simulink model "AFC_FFNN_trainbfg_15_15_15_15_Nor_July_15_RepFast"  (R2021a)
settings: Solver=ode15s  StartTime=0.0  StopTime=T  MaxStep=.01  RelTol=1e-3
undefined symbols (not defined in the file): AF_sensor_tol, fault_time, fuel_inj_tol, kappa_tol, MAF_sensor_tol, patch_sig, pump_tol, safe_patch_sig, sw, tau_ww_tol, x_gain, x_offset, y_gain, y_offset
libraries: neural x66, simulink x3
(part 1 of 3)
Description:
  | Modeling Engine Timing Using Triggered Subsystems
  | 
  | This example presents a model of a four-cylinder spark ignition engine
  | and demonstrates Simulink(R) capabilities to model an internal combustion
  | engine from the throttle to the crankshaft output. We used well-defined
  | physical principles supplemented, where appropriate, with empirical
  | relationships that describe the systems dynamic behavior without
  | introducing unnecessary complexity.
settings Model: SimulationMode=accelerator  ExtModeTrigMode=oneshot  ExtModeArmWhenConnect=off  ExtModeAutoUpdateStatusClock=off  Creator=The MathWorks Inc.  LastModifiedBy=deyun
settings SolverCC: ZeroCrossControl=DisableAll  AlgebraicLoopSolver=TrustRegion
settings DataIOCC: ExternalInput=[t__, u__]  LoadExternalInput=on  SaveFormat=StructureWithTime  SignalLogging=off  DSMLogging=off  ReturnWorkspaceOutputs=off
settings OptimizationCC: BlockReduction=off  BooleanDataType=off  LifeSpan=inf
settings DebuggingCC: SaveWithParameterizedLinksMsg=none  UnderspecifiedInitializationDetection=Classic  MergeDetectMultiDrivingBlocksExec=none  SignalResolutionControl=TryResolveAllWithWarning  ParameterPrecisionLossMsg=none  SFUnexpectedBacktrackingDiag=warning  SFNoUnconditionalDefaultTransitionDiag=warning  SFExecutionAtInitializationDiag=none  ArithmeticOperatorsInVariantConditions=warning
settings HardwareCC: ProdBitPerPointer=32  ProdBitPerSizeT=32  ProdBitPerPtrDiffT=32  ProdLargestAtomicFloat=None  ProdIntDivRoundTo=Undefined  ProdEndianess=Unspecified  ProdWordSize=32  ProdHWDeviceType=32-bit Generic  TargetBitPerLong=64  TargetBitPerPointer=64  TargetBitPerSizeT=64  TargetBitPerPtrDiffT=64  TargetLongLongMode=on  TargetIntDivRoundTo=Zero  TargetEndianess=LittleEndian  TargetWordSize=64  TargetHWDeviceType=MATLAB Host  ProdEqTarget=off
settings ModelReferenceCC: PropagateSignalLabelsOutOfModel=off
settings SFSimCC: SimUseLocalCustomCode=off  CustomCodeUndefinedFunction=UseInterfaceOnly
settings RTWCC: RTWUseLocalCustomCode=off
settings CodeAppCC: StateflowObjectComments=on
settings GRTTargetCC: TargetLangStandard=C89/C90 (ANSI)
settings ConfigComp: CovMetricSettings=d  CovSaveCumulativeToWorkspaceVar=on  CovSaveSingleToWorkspaceVar=on  CovExternalEMLEnable=off  CovBoundaryAbsTol=1.0e-5

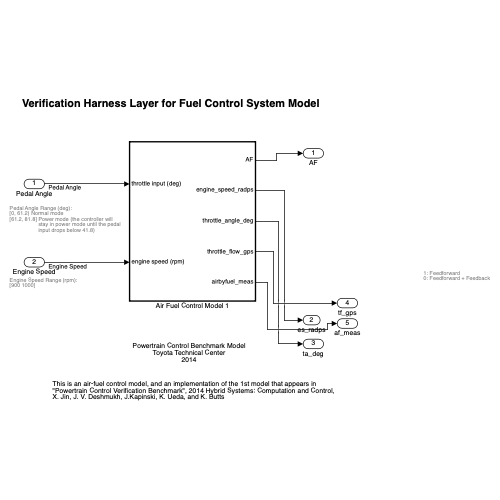
[thumbnail: Simulink's stored preview of the top-level diagram]
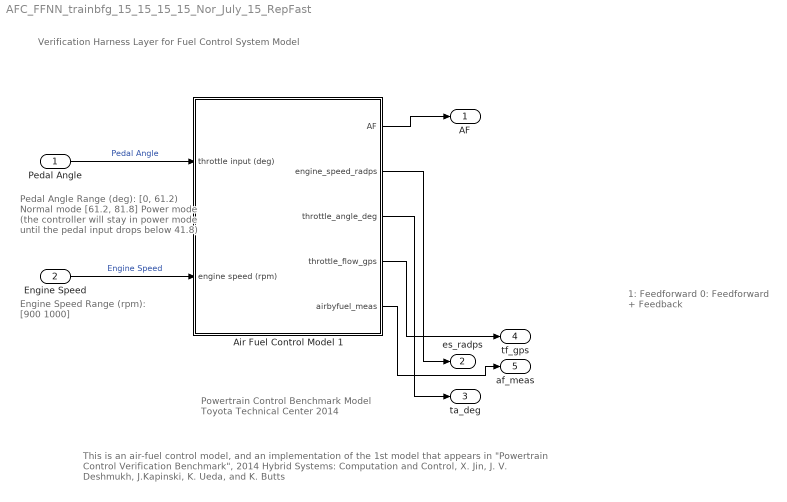
== system AFC_FFNN_trainbfg_15_15_15_15_Nor_July_15_RepFast ==
  note: 1: Feedforward
      | 0: Feedforward + Feedback
  note: Pedal Angle Range (deg):
      | [0, 61.2) Normal mode
      | [61.2, 81.8] Power mode (the controller will
      |                    stay in power mode until the pedal
      |                    input drops below 41.8)
  note: This is an air-fuel control model, and an implementation of the 1st model that appears in
      | "Powertrain Control Verification Benchmark", 2014 Hybrid Systems: Computation and Control,
      | X. Jin, J. V. Deshmukh, J.Kapinski, K. Ueda, and K. Butts
  note: Engine Speed Range (rpm):
      | [900 1000]
  note: Powertrain Control Benchmark Model
      | Toyota Technical Center
      | 2014
  note: Verification Harness Layer for Fuel Control System Model
  Pedal Angle : Inport  Interpolate=off
  Engine Speed : Inport  Port=2  Interpolate=off
  Air Fuel Control Model 1 : Subsystem  Priority=1  TreatAsAtomicUnit=on
  AF : Outport  VectorParamsAs1DForOutWhenUnconnected=off
  es_radps : Outport  Port=2
  ta_deg : Outport  Port=3
  tf_gps : Outport  Port=4
  af_meas : Outport  Port=5
  wires:
  Air Fuel Control Model 1/1(AF) -> AF/1
  Pedal Angle/1 -> Air Fuel Control Model 1/1(throttle input (deg))  "Pedal Angle"
  Engine Speed/1 -> Air Fuel Control Model 1/2(engine speed (rpm))  "Engine Speed"
  Air Fuel Control Model 1/2(engine_speed_radps) -> es_radps/1
  Air Fuel Control Model 1/3(throttle_angle_deg) -> ta_deg/1
  Air Fuel Control Model 1/4(throttle_flow_gps) -> tf_gps/1
  Air Fuel Control Model 1/5(airbyfuel_meas) -> af_meas/1

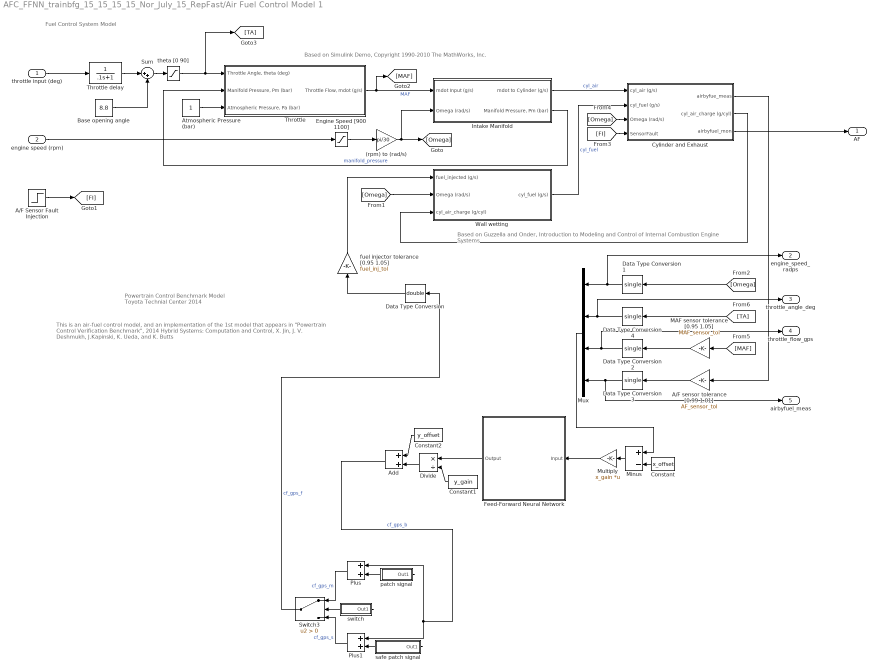
== system AFC_FFNN_trainbfg_15_15_15_15_Nor_July_15_RepFast/Air Fuel Control Model 1 ==
  note: Based on Simulink Demo, Copyright 1990-2010 The MathWorks, Inc.
  note: Based on Guzzella and Onder, Introduction to Modeling and Control of Internal Combustion Engine Systems
  note: Fuel Control System Model
  note: This is an air-fuel control model, and an implementation of the 1st model that appears in
      | "Powertrain Control Verification Benchmark", 2014 Hybrid Systems: Computation and Control,
      | X. Jin, J. V. Deshmukh, J.Kapinski, K. Ueda, and K. Butts
  note: Powertrain Control Benchmark Model
      | Toyota Technial Center
      | 2014
  throttle input (deg) : Inport  Description=[0, 81.2]
      settings: AttributesFormatString=%<Description>
  engine speed (rpm) : Inport  Description=[900,1100]  Port=2
      settings: AttributesFormatString=%<Description>
  (rpm) to (rad/s) : Gain  Gain=pi/30
  A/F Sensor Fault Injection : Step  Time=fault_time  SampleTime=0
      settings: AttributesFormatString=1: Failure\n0: Normal
  A/F sensor tolerance [0.99 1.01] : Gain  Gain=AF_sensor_tol
  Add : Sum
  Atmospheric Pressure (bar) : Constant
  Base opening angle : Constant  Value=8.8
  Constant : Constant  Value=x_offset
  Constant1 : Constant  Value=y_gain
  Constant2 : Constant  Value=y_offset
  Cylinder and Exhaust : Subsystem
  Data Type Conversion : DataTypeConversion  OutDataTypeStr=double
  Data Type Conversion{1..4} (4 alike) : DataTypeConversion  OutDataTypeStr=single
  Divide : Product  Inputs=*/
  Engine Speed [900 1100] : Saturate  UpperLimit=1100  LowerLimit=900
  Feed-Forward Neural Network : Subsystem
      mask help: Feed-Forward Neural Network
      mask Display: e = 0.06;c1 = [120 150 230]/255;c2 = ([120 150 230]+0)/383;c3 = ([120 150 230]+128)/383;patch([0 1 1 0],[0 0 1 1],c1);patch([0 1 1 1-e 1-e 0+e],[0 0 1 1-e 0+e 0+e],c2);patch([0 0 1 1-e 0+e 0+e],[0 1 1 1-e 1-e 0+e],c3);plot([0 1 1 0 0],[0 0 1 1 0]);fprintf('NNET');port_label('input',1,' Input');port_label('output',1,'Output ');
  Intake Manifold : Subsystem
  MAF sensor tolerance [0.95 1.05] : Gain  Gain=MAF_sensor_tol
  Minus : Sum  Inputs=+-
  Multiply : Gain  Gain=x_gain  Multiplication=Matrix(K*u)
  Mux : Mux
  Plus : Sum
  Plus1 : Sum
  Sum : Sum  Inputs=|++
  Switch3 : Switch  Criteria=u2 > Threshold
  Throttle : Subsystem
  Throttle delay : TransferFcn  Denominator=[.1 1]
  Wall wetting : Subsystem
  fuel injector tolerance [0.95 1.05] : Gain  Gain=fuel_inj_tol
  patch signal : Subsystem
  safe patch signal : Subsystem
  switch : Subsystem
  theta [0 90] : Saturate  UpperLimit=90  LowerLimit=0
  AF : Outport  VectorParamsAs1DForOutWhenUnconnected=off
  engine_speed_radps : Outport  Port=2
  throttle_angle_deg : Outport  Port=3
  throttle_flow_gps : Outport  Port=4
  airbyfuel_meas : Outport  Port=5
  wires:
  (rpm) to (rad/s)/1 -> [Omega], Intake Manifold/2(Omega (rad/s))
  Data Type Conversion/1 -> fuel injector tolerance [0.95 1.05]/1
  theta [0 90]/1 -> Throttle/1("Throttle Angle, theta (deg)"), [TA]
  Engine Speed [900 1100]/1 -> (rpm) to (rad/s)/1
  Cylinder and Exhaust/3("airbyfuel_mon ") -> AF/1
  A/F sensor tolerance [0.99 1.01]/1 -> Data Type Conversion3/1
  [MAF] -> MAF sensor tolerance [0.95 1.05]/1
  Cylinder and Exhaust/1(airbyfue_meas) -> A/F sensor tolerance [0.99 1.01]/1
  Throttle/1("Throttle Flow, mdot (g/s)") -> [MAF], Intake Manifold/1(mdot Input (g/s))  "MAF"
  Intake Manifold/2("Manifold Pressure, Pm (bar)") -> Throttle/2("Manifold Pressure, Pm (bar)")  "manifold_pressure"
  Atmospheric Pressure (bar)/1 -> Throttle/3("Atmospheric Pressure, Pa (bar) ")
  Wall wetting/1(cyl_fuel (g/s)) -> Cylinder and Exhaust/2(cyl_fuel (g/s))  "cyl_fuel"
  Intake Manifold/1(mdot to Cylinder (g/s)) -> Cylinder and Exhaust/1(cyl_air (g/s))  "cyl_air"
  [Omega] -> Cylinder and Exhaust/3(Omega (rad/s))
  [Omega] -> Wall wetting/2(Omega (rad/s))
  Cylinder and Exhaust/2(cyl_air_charge (g/cyl)) -> Wall wetting/3(cyl_air_charge (g/cyl))
  [Omega] -> Data Type Conversion1/1
  fuel injector tolerance [0.95 1.05]/1 -> Wall wetting/1(fuel_injected (g/s))
  MAF sensor tolerance [0.95 1.05]/1 -> Data Type Conversion2/1
  A/F Sensor Fault Injection/1 -> [FI]
  [FI] -> Cylinder and Exhaust/4(SensorFault)
  [TA] -> Data Type Conversion4/1
  throttle input (deg)/1 -> Throttle delay/1
  engine speed (rpm)/1 -> Engine Speed [900 1100]/1
  Throttle delay/1 -> Sum/1
  Base opening angle/1 -> Sum/2
  Sum/1 -> theta [0 90]/1
  Data Type Conversion3/1 -> airbyfuel_meas/1, Mux/4
  Data Type Conversion4/1 -> Mux/2, throttle_angle_deg/1
  Data Type Conversion2/1 -> Mux/3, throttle_flow_gps/1
  Data Type Conversion1/1 -> Mux/1, engine_speed_radps/1
  Multiply/1 -> Feed-Forward Neural Network/1(Input)
  Constant/1 -> Minus/2
  Mux/1 -> Minus/1
  Minus/1 -> Multiply/1
  Constant2/1 -> Add/1
  Feed-Forward Neural Network/1(Output) -> Divide/1
  Constant1/1 -> Divide/2
  Divide/1 -> Add/2
  Plus1/1 -> Switch3/3  "cf_gps_s"
  Switch3/1 -> Data Type Conversion/1  "cf_gps_f"
  Add/1 -> Plus/1, Plus1/1  "cf_gps_b"
  Plus/1 -> Switch3/1  "cf_gps_m"
  patch signal/1(Out1) -> Plus/2
  safe patch signal/1(Out1) -> Plus1/2
  switch/1(Out1) -> Switch3/2

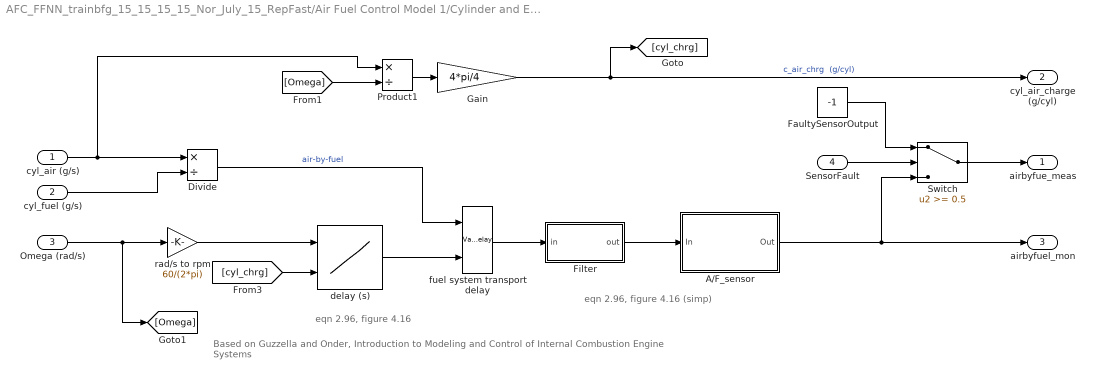
== system AFC_FFNN_trainbfg_15_15_15_15_Nor_July_15_RepFast/Air Fuel Control Model 1/Cylinder and Exhaust ==
  note: Based on Guzzella and Onder, Introduction to Modeling and Control of Internal Combustion Engine Systems
  note: eqn 2.96, figure 4.16
  note: eqn 2.96, figure 4.16 (simp)
  cyl_air (g/s) : Inport
  cyl_fuel (g/s) : Inport  Port=2
  Omega (rad/s) : Inport  Port=3
  SensorFault : Inport  Port=4
  A/F_sensor : Subsystem
  Divide : Product  Inputs=*/
  FaultySensorOutput : Constant  Value=-1
  Filter : Subsystem
  Gain : Gain  Gain=4*pi/4
  Product1 : Product  Inputs=*/  RndMeth=Zero
  Switch : Switch  Threshold=0.5
  delay (s) : Lookup_n-D  BreakpointsForDimension1=[800,1000,1500,2000,3000]  BreakpointsForDimension2=[0.05,0.15,0.2,0.25]  Table=reshape([0.8,0.6,0.4,0.3,0.2,0.4,0.3,0.2,0.2,0.2,0.3,0.25,0.2,0.2,0.2,0.25,0.2,0.2,0.2,0.2],5,4)  UseLastTableValue=on  RndMeth=Simplest  InputSameDT=on
      settings: InputPortMap=u0,u1
  fuel system transport delay : VariableTransportDelay  VariableDelayType=Variable transport delay  MaximumDelay=10  InitialOutput=14.7  MaximumPoints=20480
  rad/s to rpm : Gain  Gain=60/(2*pi)
  airbyfue_meas : Outport  VectorParamsAs1DForOutWhenUnconnected=off
  cyl_air_charge (g/cyl) : Outport  Port=2  VectorParamsAs1DForOutWhenUnconnected=off
  "airbyfuel_mon " : Outport  Port=3  VectorParamsAs1DForOutWhenUnconnected=off
  wires:
  cyl_air (g/s)/1 -> Divide/1, Product1/1
  [Omega] -> Product1/2
  Product1/1 -> Gain/1
  Gain/1 -> [cyl_chrg], cyl_air_charge (g/cyl)/1  "c_air_chrg  (g/cyl)"
  [cyl_chrg] -> delay (s)/2
  cyl_fuel (g/s)/1 -> Divide/2
  Omega (rad/s)/1 -> [Omega], rad/s to rpm/1
  rad/s to rpm/1 -> delay (s)/1
  delay (s)/1 -> fuel system transport delay/2
  fuel system transport delay/1 -> Filter/1(in)
  Switch/1 -> airbyfue_meas/1
  Divide/1 -> fuel system transport delay/1  "air-by-fuel"
  Filter/1(out) -> A/F_sensor/1(In)
  FaultySensorOutput/1 -> Switch/1
  SensorFault/1 -> Switch/2
  A/F_sensor/1(Out) -> Switch/3, "airbyfuel_mon "/1

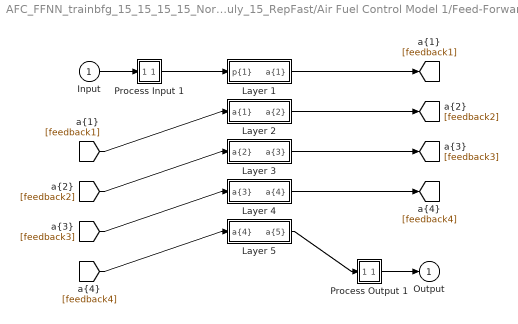
== system AFC_FFNN_trainbfg_15_15_15_15_Nor_July_15_RepFast/Air Fuel Control Model 1/Feed-Forward Neural Network ==
  Input : Inport  PortDimensions=4
      mask Display: e = 0.06;c1 = [120 230 180]/255;c2 = ([120 230 180]+0)/(256+128);c3 = ([120 230 180]+128)/(256+128);patch([0 1 1 0],[0 0 1 1],c1);patch([0 1 1 1-e 1-e 0+e],[0 0 1 1-e 0+e 0+e],c2);patch([0 0 1 1-e 0+e 0+e],[0 1 1 1-e 1-e 0+e],c3);plot([0 1 1 0 0],[0 0 1 1 0]);
  Layer 1 : Subsystem
      mask Display: e = 0.06;c1 = [120 150 230]/255;c2 = ([120 150 230]+0)/383;c3 = ([120 150 230]+128)/383;patch([0 1 1 0],[0 0 1 1],c1);patch([0 1 1 1-e 1-e 0+e],[0 0 1 1-e 0+e 0+e],c2);patch([0 0 1 1-e 0+e 0+e],[0 1 1 1-e 1-e 0+e],c3);plot([0 1 1 0 0],[0 0 1 1 0]);
  Layer 2 : Subsystem
      mask Display: e = 0.06;c1 = [120 150 230]/255;c2 = ([120 150 230]+0)/383;c3 = ([120 150 230]+128)/383;patch([0 1 1 0],[0 0 1 1],c1);patch([0 1 1 1-e 1-e 0+e],[0 0 1 1-e 0+e 0+e],c2);patch([0 0 1 1-e 0+e 0+e],[0 1 1 1-e 1-e 0+e],c3);plot([0 1 1 0 0],[0 0 1 1 0]);
  Layer 3 : Subsystem
      mask Display: e = 0.06;c1 = [120 150 230]/255;c2 = ([120 150 230]+0)/383;c3 = ([120 150 230]+128)/383;patch([0 1 1 0],[0 0 1 1],c1);patch([0 1 1 1-e 1-e 0+e],[0 0 1 1-e 0+e 0+e],c2);patch([0 0 1 1-e 0+e 0+e],[0 1 1 1-e 1-e 0+e],c3);plot([0 1 1 0 0],[0 0 1 1 0]);
  Layer 4 : Subsystem
      mask Display: e = 0.06;c1 = [120 150 230]/255;c2 = ([120 150 230]+0)/383;c3 = ([120 150 230]+128)/383;patch([0 1 1 0],[0 0 1 1],c1);patch([0 1 1 1-e 1-e 0+e],[0 0 1 1-e 0+e 0+e],c2);patch([0 0 1 1-e 0+e 0+e],[0 1 1 1-e 1-e 0+e],c3);plot([0 1 1 0 0],[0 0 1 1 0]);
  Layer 5 : Subsystem
      mask Display: e = 0.06;c1 = [120 150 230]/255;c2 = ([120 150 230]+0)/383;c3 = ([120 150 230]+128)/383;patch([0 1 1 0],[0 0 1 1],c1);patch([0 1 1 1-e 1-e 0+e],[0 0 1 1-e 0+e 0+e],c2);patch([0 0 1 1-e 0+e 0+e],[0 1 1 1-e 1-e 0+e],c3);plot([0 1 1 0 0],[0 0 1 1 0]);
  Process Input 1 : Subsystem
      mask Display: e = 0.06;c1 = [120 150 230]/255;c2 = ([120 150 230]+0)/383;c3 = ([120 150 230]+128)/383;patch([0 1 1 0],[0 0 1 1],c1);patch([0 1 1 1-e 1-e 0+e],[0 0 1 1-e 0+e 0+e],c2);patch([0 0 1 1-e 0+e 0+e],[0 1 1 1-e 1-e 0+e],c3);plot([0 1 1 0 0],[0 0 1 1 0]);
  Process Output 1 : Subsystem
      mask Display: e = 0.06;c1 = [120 150 230]/255;c2 = ([120 150 230]+0)/383;c3 = ([120 150 230]+128)/383;patch([0 1 1 0],[0 0 1 1],c1);patch([0 1 1 1-e 1-e 0+e],[0 0 1 1-e 0+e 0+e],c2);patch([0 0 1 1-e 0+e 0+e],[0 1 1 1-e 1-e 0+e],c3);plot([0 1 1 0 0],[0 0 1 1 0]);
  Output : Outport  InitialOutput=0
      mask Display: e = 0.06;c1 = [120 230 180]/255;c2 = ([120 230 180]+0)/(256+128);c3 = ([120 230 180]+128)/(256+128);patch([0 1 1 0],[0 0 1 1],c1);patch([0 1 1 1-e 1-e 0+e],[0 0 1 1-e 0+e 0+e],c2);patch([0 0 1 1-e 0+e 0+e],[0 1 1 1-e 1-e 0+e],c3);plot([0 1 1 0 0],[0 0 1 1 0]);
  wires:
  Layer 5/1("a{5}") -> Process Output 1/1(a)
  [feedback4] -> Layer 5/1("a{4} ")
  Layer 4/1("a{4}") -> [feedback4]
  [feedback3] -> Layer 4/1("a{3} ")
  Layer 3/1("a{3}") -> [feedback3]
  [feedback2] -> Layer 3/1("a{2} ")
  Layer 2/1("a{2}") -> [feedback2]
  [feedback1] -> Layer 2/1("a{1} ")
  Layer 1/1("a{1}") -> [feedback1]
  Process Input 1/1(p) -> Layer 1/1("p{1}")
  Process Output 1/1(y) -> Output/1
  Input/1 -> Process Input 1/1(x)

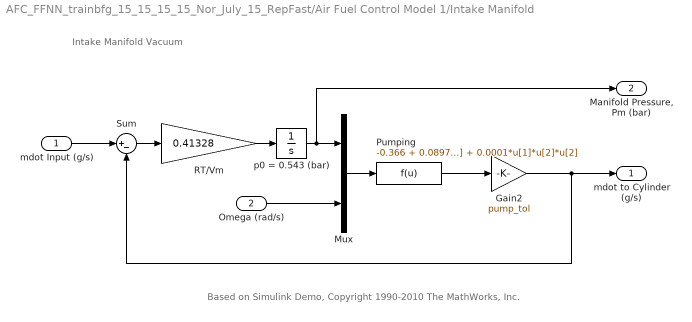
== system AFC_FFNN_trainbfg_15_15_15_15_Nor_July_15_RepFast/Air Fuel Control Model 1/Intake Manifold ==
  note: Intake Manifold Vacuum
  note: Based on Simulink Demo, Copyright 1990-2010 The MathWorks, Inc.
  mdot Input (g/s) : Inport
  Omega (rad/s) : Inport  Port=2
  Gain2 : Gain  Gain=pump_tol  ParamDataTypeStr=single  OutDataTypeStr=Inherit: Inherit via back propagation  RndMeth=Simplest  SaturateOnIntegerOverflow=on
      settings: AttributesFormatString=pumping tolerance [0.9 1.1]
  Mux : Mux  Inputs=2
  Pumping : Fcn  Expr=-0.366 + 0.08979*u[1]*u[2] - 0.0337*u[2]*u[1]*u[1] + 0.0001*u[1]*u[2]*u[2]
  RT/Vm : Gain  Gain=0.41328  SaturateOnIntegerOverflow=on  OutDataTypeStr=Inherit: Same as input  ParamDataTypeStr=Inherit: Same as input
  Sum : Sum  Inputs=|+-  InputSameDT=on  SaturateOnIntegerOverflow=on  OutDataTypeStr=Inherit: Same as first input
  p0 = 0.543 (bar) : Integrator  InitialCondition=0.982
  mdot to Cylinder (g/s) : Outport  InitialOutput=0  VectorParamsAs1DForOutWhenUnconnected=off
  "Manifold Pressure, Pm (bar)" : Outport  Port=2  InitialOutput=0  VectorParamsAs1DForOutWhenUnconnected=off
  wires:
  mdot Input (g/s)/1 -> Sum/1
  RT/Vm/1 -> p0 = 0.543 (bar)/1
  Omega (rad/s)/1 -> Mux/2
  Mux/1 -> Pumping/1
  p0 = 0.543 (bar)/1 -> Mux/1, "Manifold Pressure, Pm (bar)"/1
  Sum/1 -> RT/Vm/1
  Pumping/1 -> Gain2/1
  Gain2/1 -> Sum/2, mdot to Cylinder (g/s)/1

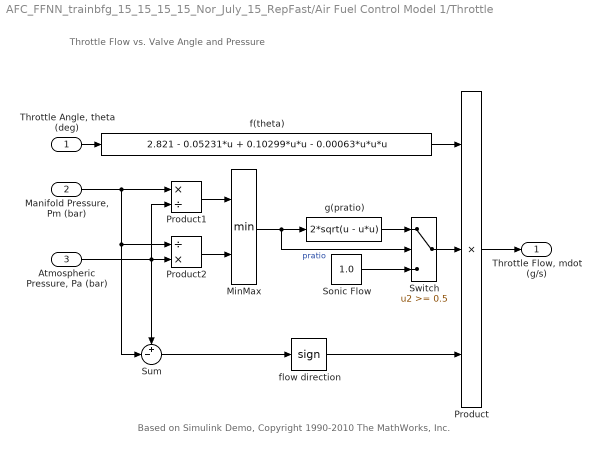
== system AFC_FFNN_trainbfg_15_15_15_15_Nor_July_15_RepFast/Air Fuel Control Model 1/Throttle ==
  note: Throttle Flow vs. Valve Angle and Pressure
  note: Based on Simulink Demo, Copyright 1990-2010 The MathWorks, Inc.
  "Throttle Angle, theta (deg)" : Inport
  "Manifold Pressure, Pm (bar)" : Inport  Port=2
  "Atmospheric Pressure, Pa (bar) " : Inport  Port=3
  MinMax : MinMax  Inputs=2  InputSameDT=on  SaturateOnIntegerOverflow=on
  Product : Product  Inputs=3  InputSameDT=on  RndMeth=Zero  SaturateOnIntegerOverflow=on  OutDataTypeStr=Inherit: Same as first input
  Product1 : Product  Inputs=*/  InputSameDT=on  RndMeth=Zero  SaturateOnIntegerOverflow=on  OutDataTypeStr=Inherit: Same as first input
  Product2 : Product  Inputs=/*  InputSameDT=on  RndMeth=Zero  SaturateOnIntegerOverflow=on  OutDataTypeStr=Inherit: Same as first input
  "Sonic Flow " : Constant  Value=1.0
  Sum : Sum  Inputs=+-|  InputSameDT=on  SaturateOnIntegerOverflow=on  OutDataTypeStr=Inherit: Same as first input
  Switch : Switch  Threshold=0.5  SaturateOnIntegerOverflow=on  InputSameDT=on
  f(theta) : Fcn  Expr=2.821 - 0.05231*u + 0.10299*u*u - 0.00063*u*u*u
  flow direction : Signum
  g(pratio) : Fcn  Expr=2*sqrt(u - u*u)
  "Throttle Flow, mdot (g/s)" : Outport  InitialOutput=0  VectorParamsAs1DForOutWhenUnconnected=off
  wires:
  "Manifold Pressure, Pm (bar)"/1 -> Sum/2, Product2/1, Product1/1
  Product2/1 -> MinMax/2
  Product1/1 -> MinMax/1
  "Atmospheric Pressure, Pa (bar) "/1 -> Sum/1, Product2/2, Product1/2
  g(pratio)/1 -> Switch/1
  "Sonic Flow "/1 -> Switch/3
  Switch/1 -> Product/2
  flow direction/1 -> Product/3
  Sum/1 -> flow direction/1
  MinMax/1 -> g(pratio)/1, Switch/2  "pratio"
  "Throttle Angle, theta (deg)"/1 -> f(theta)/1
  Product/1 -> "Throttle Flow, mdot (g/s)"/1
  f(theta)/1 -> Product/1

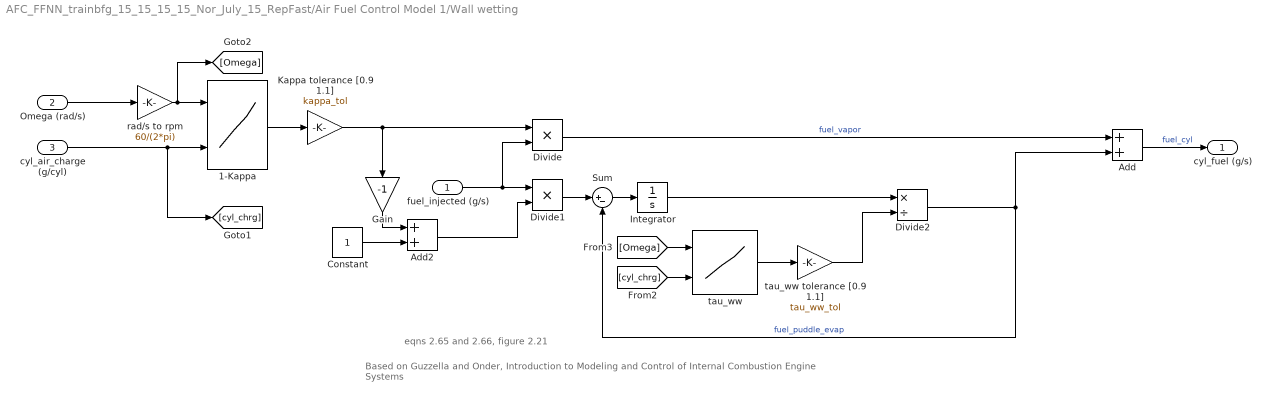
== system AFC_FFNN_trainbfg_15_15_15_15_Nor_July_15_RepFast/Air Fuel Control Model 1/Wall wetting ==
  note: Based on Guzzella and Onder, Introduction to Modeling and Control of Internal Combustion Engine Systems
  note: eqns 2.65 and 2.66, figure 2.21
  fuel_injected (g/s) : Inport
  Omega (rad/s) : Inport  Port=2
  cyl_air_charge (g/cyl) : Inport  Port=3
  1-Kappa : Lookup_n-D  BreakpointsForDimension1=[1000,1500,2000,2500,3000]  BreakpointsForDimension2=[.1,.2,.3,.4]  Table=reshape([0.8,.7,.7,.8,.9,.7,.66,.65,.73,.85,.66,.66,.63,.66,.8,.6,.6,.6,.6,.7],5,4)  UseLastTableValue=on  RndMeth=Simplest  InputSameDT=on
      settings: InputPortMap=u0,u1
  Add : Sum
  Add2 : Sum
  Constant : Constant
  Divide : Product  Inputs=**
  Divide1 : Product  Inputs=**
  Divide2 : Product  Inputs=*/
  Gain : Gain  Gain=-1
  Integrator : Integrator  InitialCondition=.0112
  Kappa tolerance [0.9 1.1] : Gain  Gain=kappa_tol
  Sum : Sum  Inputs=|+-
  rad/s to rpm : Gain  Gain=60/(2*pi)
  tau_ww : Lookup_n-D  BreakpointsForDimension1=[1000,1500,2000,2500,3000]  BreakpointsForDimension2=[0.1,0.2,0.3,0.4]  Table=reshape([.4,.3,.35,.3,.2,.22,.22,.4,.35,.5,.20,.22,.5,.4,.35,.35,.3,.45,.5,.4],5,4)  UseLastTableValue=on  RndMeth=Simplest  InputSameDT=on
      settings: InputPortMap=u0,u1
  tau_ww tolerance [0.9 1.1] : Gain  Gain=tau_ww_tol
  cyl_fuel (g/s) : Outport  VectorParamsAs1DForOutWhenUnconnected=off
  wires:
  1-Kappa/1 -> Kappa tolerance [0.9 1.1]/1
  fuel_injected (g/s)/1 -> Divide/2, Divide1/1
  Divide/1 -> Add/1  "fuel_vapor"
  Add/1 -> cyl_fuel (g/s)/1  "fuel_cyl"
  Integrator/1 -> Divide2/1
  Divide1/1 -> Sum/1
  Sum/1 -> Integrator/1
  Divide2/1 -> Add/2, Sum/2  "fuel_puddle_evap"
  Add2/1 -> Divide1/2
  cyl_air_charge (g/cyl)/1 -> 1-Kappa/2, [cyl_chrg]
  [cyl_chrg] -> tau_ww/2
  tau_ww/1 -> tau_ww tolerance [0.9 1.1]/1
  Gain/1 -> Add2/1
  Constant/1 -> Add2/2
  rad/s to rpm/1 -> [Omega], 1-Kappa/1
  Omega (rad/s)/1 -> rad/s to rpm/1
  Kappa tolerance [0.9 1.1]/1 -> Divide/1, Gain/1
  tau_ww tolerance [0.9 1.1]/1 -> Divide2/2
  [Omega] -> tau_ww/1

== system AFC_FFNN_trainbfg_15_15_15_15_Nor_July_15_RepFast/Air Fuel Control Model 1/patch signal ==
  Sample index : simulink/Sources/Counter Limited  uplimit=numel(patch_sig)-1  tsamp=Ts
  Sample value : LookupNDDirect  NumberOfTableDimensions=1  Table=patch_sig  DiagnosticForOutOfRangeInput=None
  Out1 : Outport
  wires:
  Sample index/1 -> Sample value/1
  Sample value/1 -> Out1/1

== system AFC_FFNN_trainbfg_15_15_15_15_Nor_July_15_RepFast/Air Fuel Control Model 1/safe patch signal ==
  Sample index : simulink/Sources/Counter Limited  uplimit=numel(safe_patch_sig)-1  tsamp=Ts
  Sample value : LookupNDDirect  NumberOfTableDimensions=1  Table=safe_patch_sig  DiagnosticForOutOfRangeInput=None
  Out1 : Outport
  wires:
  Sample index/1 -> Sample value/1
  Sample value/1 -> Out1/1

== system AFC_FFNN_trainbfg_15_15_15_15_Nor_July_15_RepFast/Air Fuel Control Model 1/switch ==
  Sample index : simulink/Sources/Counter Limited  uplimit=numel(sw)-1  tsamp=Ts
  Sample value : LookupNDDirect  NumberOfTableDimensions=1  Table=sw  DiagnosticForOutOfRangeInput=None
  Out1 : Outport
  wires:
  Sample index/1 -> Sample value/1
  Sample value/1 -> Out1/1

== system AFC_FFNN_trainbfg_15_15_15_15_Nor_July_15_RepFast/Air Fuel Control Model 1/Cylinder and Exhaust/A//F_sensor ==
  In : Inport
  A/F_sensor : Gain  OutDataTypeStr=double
  Filter : Subsystem
  Out : Outport  VectorParamsAs1DForOutWhenUnconnected=off
  wires:
  A/F_sensor/1 -> Out/1
  In/1 -> Filter/1(In)
  Filter/1(Out) -> A/F_sensor/1

== system AFC_FFNN_trainbfg_15_15_15_15_Nor_July_15_RepFast/Air Fuel Control Model 1/Cylinder and Exhaust/Filter ==
  in : Inport
  Gain1 : Gain  Gain=10
  Integrator : Integrator  InitialCondition=14.7
  Sum : Sum  Inputs=|+-
  out : Outport  VectorParamsAs1DForOutWhenUnconnected=off
  wires:
  Integrator/1 -> out/1, Sum/2
  in/1 -> Sum/1
  Gain1/1 -> Integrator/1
  Sum/1 -> Gain1/1

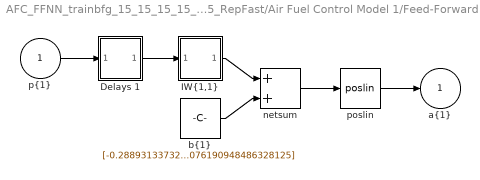
== system AFC_FFNN_trainbfg_15_15_15_15_Nor_July_15_RepFast/Air Fuel Control Model 1/Feed-Forward Neural Network/Layer 1 ==
  "p{1}" : Inport  PortDimensions=4
      mask Display: e = 0.06;c1 = [120 230 180]/255;c2 = ([120 230 180]+0)/(256+128);c3 = ([120 230 180]+128)/(256+128);patch([0 1 1 0],[0 0 1 1],c1);patch([0 1 1 1-e 1-e 0+e],[0 0 1 1-e 0+e 0+e],c2);patch([0 0 1 1-e 0+e 0+e],[0 1 1 1-e 1-e 0+e],c3);plot([0 1 1 0 0],[0 0 1 1 0]);
  Delays 1 : Subsystem
      mask Display: e = 0.06;c1 = [120 150 230]/255;c2 = ([120 150 230]+0)/383;c3 = ([120 150 230]+128)/383;patch([0 1 1 0],[0 0 1 1],c1);patch([0 1 1 1-e 1-e 0+e],[0 0 1 1-e 0+e 0+e],c2);patch([0 0 1 1-e 0+e 0+e],[0 1 1 1-e 1-e 0+e],c3);plot([0 1 1 0 0],[0 0 1 1 0]);disp('0');
  "IW{1,1}" : Subsystem
      mask Display: e = 0.06;c1 = [120 150 230]/255;c2 = ([120 150 230]+0)/383;c3 = ([120 150 230]+128)/383;patch([0 1 1 0],[0 0 1 1],c1);patch([0 1 1 1-e 1-e 0+e],[0 0 1 1-e 0+e 0+e],c2);patch([0 0 1 1-e 0+e 0+e],[0 1 1 1-e 1-e 0+e],c3);plot([0 1 1 0 0],[0 0 1 1 0]);disp('W');
  "b{1}" : Constant  Value=[-0.2889313373298836307156989278155378997325897216796875;-0.6859020619533524598665508165140636265277862548828125;-0.5776774272060449799681691729347221553325653076171875;1.0962588133114949950908112441538833081722259521484375;-0.347378437377750814984977978383540175855159759521484375;-0.81669590775078260147523678824654780328273773193359375;-0.798278791842729873451389721594750881195068359375;-0.8415000061570527822851772725698538124561309814453125;-0.93301053623252894198003559722565114498138427734375;-1.187779921006250294368555842083878815174102783203125;-0.71550410350406623560814978191046975553035736083984375;1.5443917967751108477614252478815615177154541015625;2.491113182252983282438663081848062574863433837890625;2.559427572241828041654798653325997292995452880859375;-0.72959281569020106861245267282356508076190948486328125]
      mask Display: e = 0.06;c1 = [120 150 230]/255;c2 = ([120 150 230]+0)/383;c3 = ([120 150 230]+128)/383;patch([0 1 1 0],[0 0 1 1],c1);patch([0 1 1 1-e 1-e 0+e],[0 0 1 1-e 0+e 0+e],c2);patch([0 0 1 1-e 0+e 0+e],[0 1 1 1-e 1-e 0+e],c3);plot([0 1 1 0 0],[0 0 1 1 0]);disp('b');
  netsum : Sum  Inputs=2  InputSameDT=on  SaturateOnIntegerOverflow=on  OutDataTypeStr=Inherit: Same as first input
      mask Display: e = 0.06;c1 = [120 150 230]/255;c2 = ([120 150 230]+0)/383;c3 = ([120 150 230]+128)/383;patch([0 1 1 0],[0 0 1 1],c1);patch([0 1 1 1-e 1-e 0+e],[0 0 1 1-e 0+e 0+e],c2);patch([0 0 1 1-e 0+e 0+e],[0 1 1 1-e 1-e 0+e],c3);plot([0 1 1 0 0],[0 0 1 1 0]);disp('+');
  poslin : neural/Transfer Functions/poslin
  "a{1}" : Outport  InitialOutput=[0;0;0;0;0;0;0;0;0;0;0;0;0;0;0]
      mask Display: e = 0.06;c1 = [120 230 180]/255;c2 = ([120 230 180]+0)/(256+128);c3 = ([120 230 180]+128)/(256+128);patch([0 1 1 0],[0 0 1 1],c1);patch([0 1 1 1-e 1-e 0+e],[0 0 1 1-e 0+e 0+e],c2);patch([0 0 1 1-e 0+e 0+e],[0 1 1 1-e 1-e 0+e],c3);plot([0 1 1 0 0],[0 0 1 1 0]);
  wires:
  poslin/1 -> "a{1}"/1
  netsum/1 -> poslin/1
  "b{1}"/1 -> netsum/2
  "IW{1,1}"/1("iz{1,1}") -> netsum/1
  Delays 1/1("pd{1,1}") -> "IW{1,1}"/1("pd{1,1}")
  "p{1}"/1 -> Delays 1/1("p{1}")

== system AFC_FFNN_trainbfg_15_15_15_15_Nor_July_15_RepFast/Air Fuel Control Model 1/Feed-Forward Neural Network/Layer 2 ==
  "a{1} " : Inport  PortDimensions=15
      mask Display: e = 0.06;c1 = [120 230 180]/255;c2 = ([120 230 180]+0)/(256+128);c3 = ([120 230 180]+128)/(256+128);patch([0 1 1 0],[0 0 1 1],c1);patch([0 1 1 1-e 1-e 0+e],[0 0 1 1-e 0+e 0+e],c2);patch([0 0 1 1-e 0+e 0+e],[0 1 1 1-e 1-e 0+e],c3);plot([0 1 1 0 0],[0 0 1 1 0]);
  Delays 1 : Subsystem
      mask Display: e = 0.06;c1 = [120 150 230]/255;c2 = ([120 150 230]+0)/383;c3 = ([120 150 230]+128)/383;patch([0 1 1 0],[0 0 1 1],c1);patch([0 1 1 1-e 1-e 0+e],[0 0 1 1-e 0+e 0+e],c2);patch([0 0 1 1-e 0+e 0+e],[0 1 1 1-e 1-e 0+e],c3);plot([0 1 1 0 0],[0 0 1 1 0]);disp('0');
  "LW{2,1}" : Subsystem
      mask Display: e = 0.06;c1 = [120 150 230]/255;c2 = ([120 150 230]+0)/383;c3 = ([120 150 230]+128)/383;patch([0 1 1 0],[0 0 1 1],c1);patch([0 1 1 1-e 1-e 0+e],[0 0 1 1-e 0+e 0+e],c2);patch([0 0 1 1-e 0+e 0+e],[0 1 1 1-e 1-e 0+e],c3);plot([0 1 1 0 0],[0 0 1 1 0]);disp('W');
  "b{2}" : Constant  Value=[-0.268014232209020430985901839449070394039154052734375;0.1493455357010621542546147111352183856070041656494140625;-0.49746015489066219839031646188232116401195526123046875;0.72945240731106253395665817151893861591815948486328125;-0.72251921283007281004984179162420332431793212890625;0.1678413393382454932289959970148629508912563323974609375;-0.39488807769449607576461858116090297698974609375;0.4534437848455354913568271513213403522968292236328125;0.157254173389736295884944183853804133832454681396484375;-0.402355228407594911477218602158245630562305450439453125;-0.5069072823348392820008712078561075031757354736328125;-0.7993983612316426512478528820793144404888153076171875;-0.326427311408129583458759270797600038349628448486328125;-2.01503583284488829718839042470790445804595947265625;0.22673419984890352818496239706291817128658294677734375]
      mask Display: e = 0.06;c1 = [120 150 230]/255;c2 = ([120 150 230]+0)/383;c3 = ([120 150 230]+128)/383;patch([0 1 1 0],[0 0 1 1],c1);patch([0 1 1 1-e 1-e 0+e],[0 0 1 1-e 0+e 0+e],c2);patch([0 0 1 1-e 0+e 0+e],[0 1 1 1-e 1-e 0+e],c3);plot([0 1 1 0 0],[0 0 1 1 0]);disp('b');
  netsum : Sum  Inputs=2  InputSameDT=on  SaturateOnIntegerOverflow=on  OutDataTypeStr=Inherit: Same as first input
      mask Display: e = 0.06;c1 = [120 150 230]/255;c2 = ([120 150 230]+0)/383;c3 = ([120 150 230]+128)/383;patch([0 1 1 0],[0 0 1 1],c1);patch([0 1 1 1-e 1-e 0+e],[0 0 1 1-e 0+e 0+e],c2);patch([0 0 1 1-e 0+e 0+e],[0 1 1 1-e 1-e 0+e],c3);plot([0 1 1 0 0],[0 0 1 1 0]);disp('+');
  poslin : neural/Transfer Functions/poslin
  "a{2}" : Outport  InitialOutput=[0;0;0;0;0;0;0;0;0;0;0;0;0;0;0]
      mask Display: e = 0.06;c1 = [120 230 180]/255;c2 = ([120 230 180]+0)/(256+128);c3 = ([120 230 180]+128)/(256+128);patch([0 1 1 0],[0 0 1 1],c1);patch([0 1 1 1-e 1-e 0+e],[0 0 1 1-e 0+e 0+e],c2);patch([0 0 1 1-e 0+e 0+e],[0 1 1 1-e 1-e 0+e],c3);plot([0 1 1 0 0],[0 0 1 1 0]);
  wires:
  poslin/1 -> "a{2}"/1
  netsum/1 -> poslin/1
  "b{2}"/1 -> netsum/2
  "LW{2,1}"/1("lz{2,1}") -> netsum/1
  Delays 1/1("pd{2,1}") -> "LW{2,1}"/1("ad{2,1}")
  "a{1} "/1 -> Delays 1/1("p{2}")

== system AFC_FFNN_trainbfg_15_15_15_15_Nor_July_15_RepFast/Air Fuel Control Model 1/Feed-Forward Neural Network/Layer 3 ==
  "a{2} " : Inport  PortDimensions=15
      mask Display: e = 0.06;c1 = [120 230 180]/255;c2 = ([120 230 180]+0)/(256+128);c3 = ([120 230 180]+128)/(256+128);patch([0 1 1 0],[0 0 1 1],c1);patch([0 1 1 1-e 1-e 0+e],[0 0 1 1-e 0+e 0+e],c2);patch([0 0 1 1-e 0+e 0+e],[0 1 1 1-e 1-e 0+e],c3);plot([0 1 1 0 0],[0 0 1 1 0]);
  Delays 1 : Subsystem
      mask Display: e = 0.06;c1 = [120 150 230]/255;c2 = ([120 150 230]+0)/383;c3 = ([120 150 230]+128)/383;patch([0 1 1 0],[0 0 1 1],c1);patch([0 1 1 1-e 1-e 0+e],[0 0 1 1-e 0+e 0+e],c2);patch([0 0 1 1-e 0+e 0+e],[0 1 1 1-e 1-e 0+e],c3);plot([0 1 1 0 0],[0 0 1 1 0]);disp('0');
  "LW{3,2}" : Subsystem
      mask Display: e = 0.06;c1 = [120 150 230]/255;c2 = ([120 150 230]+0)/383;c3 = ([120 150 230]+128)/383;patch([0 1 1 0],[0 0 1 1],c1);patch([0 1 1 1-e 1-e 0+e],[0 0 1 1-e 0+e 0+e],c2);patch([0 0 1 1-e 0+e 0+e],[0 1 1 1-e 1-e 0+e],c3);plot([0 1 1 0 0],[0 0 1 1 0]);disp('W');
  "b{3}" : Constant  Value=[0.362863840056467268357920374910463578999042510986328125;-0.88172590754745405750014697332517243921756744384765625;0.06590743028277541715187481941029545851051807403564453125;-0.757556142707523694213023190968669950962066650390625;-0.88366778143589652660949695928138680756092071533203125;0.8273911823557520417438126969500444829463958740234375;-0.487685738531727253075587213970720767974853515625;0.4714966042974941817789158449159003794193267822265625;-0.24727281081949659125029938877560198307037353515625;-0.52279692926543763764613004241255111992359161376953125;0.1077342921915615814310029918487998656928539276123046875;1.141151155229312319505652340012602508068084716796875;-0.0611236831323188900544352009092108346521854400634765625;0.6368889963582018420851227347156964242458343505859375;0.929420783334013123067052219994366168975830078125]
      mask Display: e = 0.06;c1 = [120 150 230]/255;c2 = ([120 150 230]+0)/383;c3 = ([120 150 230]+128)/383;patch([0 1 1 0],[0 0 1 1],c1);patch([0 1 1 1-e 1-e 0+e],[0 0 1 1-e 0+e 0+e],c2);patch([0 0 1 1-e 0+e 0+e],[0 1 1 1-e 1-e 0+e],c3);plot([0 1 1 0 0],[0 0 1 1 0]);disp('b');
  netsum : Sum  Inputs=2  InputSameDT=on  SaturateOnIntegerOverflow=on  OutDataTypeStr=Inherit: Same as first input
      mask Display: e = 0.06;c1 = [120 150 230]/255;c2 = ([120 150 230]+0)/383;c3 = ([120 150 230]+128)/383;patch([0 1 1 0],[0 0 1 1],c1);patch([0 1 1 1-e 1-e 0+e],[0 0 1 1-e 0+e 0+e],c2);patch([0 0 1 1-e 0+e 0+e],[0 1 1 1-e 1-e 0+e],c3);plot([0 1 1 0 0],[0 0 1 1 0]);disp('+');
  poslin : neural/Transfer Functions/poslin
  "a{3}" : Outport  InitialOutput=[0;0;0;0;0;0;0;0;0;0;0;0;0;0;0]
      mask Display: e = 0.06;c1 = [120 230 180]/255;c2 = ([120 230 180]+0)/(256+128);c3 = ([120 230 180]+128)/(256+128);patch([0 1 1 0],[0 0 1 1],c1);patch([0 1 1 1-e 1-e 0+e],[0 0 1 1-e 0+e 0+e],c2);patch([0 0 1 1-e 0+e 0+e],[0 1 1 1-e 1-e 0+e],c3);plot([0 1 1 0 0],[0 0 1 1 0]);
  wires:
  poslin/1 -> "a{3}"/1
  netsum/1 -> poslin/1
  "b{3}"/1 -> netsum/2
  "LW{3,2}"/1("lz{3,2}") -> netsum/1
  Delays 1/1("pd{3,2}") -> "LW{3,2}"/1("ad{3,2}")
  "a{2} "/1 -> Delays 1/1("p{3}")

== system AFC_FFNN_trainbfg_15_15_15_15_Nor_July_15_RepFast/Air Fuel Control Model 1/Feed-Forward Neural Network/Layer 4 ==
  "a{3} " : Inport  PortDimensions=15
      mask Display: e = 0.06;c1 = [120 230 180]/255;c2 = ([120 230 180]+0)/(256+128);c3 = ([120 230 180]+128)/(256+128);patch([0 1 1 0],[0 0 1 1],c1);patch([0 1 1 1-e 1-e 0+e],[0 0 1 1-e 0+e 0+e],c2);patch([0 0 1 1-e 0+e 0+e],[0 1 1 1-e 1-e 0+e],c3);plot([0 1 1 0 0],[0 0 1 1 0]);
  Delays 1 : Subsystem
      mask Display: e = 0.06;c1 = [120 150 230]/255;c2 = ([120 150 230]+0)/383;c3 = ([120 150 230]+128)/383;patch([0 1 1 0],[0 0 1 1],c1);patch([0 1 1 1-e 1-e 0+e],[0 0 1 1-e 0+e 0+e],c2);patch([0 0 1 1-e 0+e 0+e],[0 1 1 1-e 1-e 0+e],c3);plot([0 1 1 0 0],[0 0 1 1 0]);disp('0');
  "LW{4,3}" : Subsystem
      mask Display: e = 0.06;c1 = [120 150 230]/255;c2 = ([120 150 230]+0)/383;c3 = ([120 150 230]+128)/383;patch([0 1 1 0],[0 0 1 1],c1);patch([0 1 1 1-e 1-e 0+e],[0 0 1 1-e 0+e 0+e],c2);patch([0 0 1 1-e 0+e 0+e],[0 1 1 1-e 1-e 0+e],c3);plot([0 1 1 0 0],[0 0 1 1 0]);disp('W');
  "b{4}" : Constant  Value=[-0.474809754705890540993351578435976989567279815673828125;-0.0976772386611539644718504860065877437591552734375;-0.004470636884659269505437606539999251253902912139892578125;-0.7269848601738202464872529162676073610782623291015625;0.287303918106255162800977132064872421324253082275390625;-0.8985667154179868276742126909084618091583251953125;0.5320032594627244204588123466237448155879974365234375;-0.919593644113579689047810461488552391529083251953125;0.398808301712129276150875512030324898660182952880859375;-0.89306373672204941716046278088469989597797393798828125;0.2214065631604686668065795629445347003638744354248046875;0.2712440384256302738918975592241622507572174072265625;-0.59897319160038653418354215318686328828334808349609375;0.67968471746184722093175878399051725864410400390625;-0.26409910243741119284521801091614179313182830810546875]
      mask Display: e = 0.06;c1 = [120 150 230]/255;c2 = ([120 150 230]+0)/383;c3 = ([120 150 230]+128)/383;patch([0 1 1 0],[0 0 1 1],c1);patch([0 1 1 1-e 1-e 0+e],[0 0 1 1-e 0+e 0+e],c2);patch([0 0 1 1-e 0+e 0+e],[0 1 1 1-e 1-e 0+e],c3);plot([0 1 1 0 0],[0 0 1 1 0]);disp('b');
  netsum : Sum  Inputs=2  InputSameDT=on  SaturateOnIntegerOverflow=on  OutDataTypeStr=Inherit: Same as first input
      mask Display: e = 0.06;c1 = [120 150 230]/255;c2 = ([120 150 230]+0)/383;c3 = ([120 150 230]+128)/383;patch([0 1 1 0],[0 0 1 1],c1);patch([0 1 1 1-e 1-e 0+e],[0 0 1 1-e 0+e 0+e],c2);patch([0 0 1 1-e 0+e 0+e],[0 1 1 1-e 1-e 0+e],c3);plot([0 1 1 0 0],[0 0 1 1 0]);disp('+');
  poslin : neural/Transfer Functions/poslin
  "a{4}" : Outport  InitialOutput=[0;0;0;0;0;0;0;0;0;0;0;0;0;0;0]
      mask Display: e = 0.06;c1 = [120 230 180]/255;c2 = ([120 230 180]+0)/(256+128);c3 = ([120 230 180]+128)/(256+128);patch([0 1 1 0],[0 0 1 1],c1);patch([0 1 1 1-e 1-e 0+e],[0 0 1 1-e 0+e 0+e],c2);patch([0 0 1 1-e 0+e 0+e],[0 1 1 1-e 1-e 0+e],c3);plot([0 1 1 0 0],[0 0 1 1 0]);
  wires:
  poslin/1 -> "a{4}"/1
  netsum/1 -> poslin/1
  "b{4}"/1 -> netsum/2
  "LW{4,3}"/1("lz{4,3}") -> netsum/1
  Delays 1/1("pd{4,3}") -> "LW{4,3}"/1("ad{4,3}")
  "a{3} "/1 -> Delays 1/1("p{4}")

== system AFC_FFNN_trainbfg_15_15_15_15_Nor_July_15_RepFast/Air Fuel Control Model 1/Feed-Forward Neural Network/Layer 5 ==
  "a{4} " : Inport  PortDimensions=15
      mask Display: e = 0.06;c1 = [120 230 180]/255;c2 = ([120 230 180]+0)/(256+128);c3 = ([120 230 180]+128)/(256+128);patch([0 1 1 0],[0 0 1 1],c1);patch([0 1 1 1-e 1-e 0+e],[0 0 1 1-e 0+e 0+e],c2);patch([0 0 1 1-e 0+e 0+e],[0 1 1 1-e 1-e 0+e],c3);plot([0 1 1 0 0],[0 0 1 1 0]);
  Delays 1 : Subsystem
      mask Display: e = 0.06;c1 = [120 150 230]/255;c2 = ([120 150 230]+0)/383;c3 = ([120 150 230]+128)/383;patch([0 1 1 0],[0 0 1 1],c1);patch([0 1 1 1-e 1-e 0+e],[0 0 1 1-e 0+e 0+e],c2);patch([0 0 1 1-e 0+e 0+e],[0 1 1 1-e 1-e 0+e],c3);plot([0 1 1 0 0],[0 0 1 1 0]);disp('0');
  "LW{5,4}" : Subsystem
      mask Display: e = 0.06;c1 = [120 150 230]/255;c2 = ([120 150 230]+0)/383;c3 = ([120 150 230]+128)/383;patch([0 1 1 0],[0 0 1 1],c1);patch([0 1 1 1-e 1-e 0+e],[0 0 1 1-e 0+e 0+e],c2);patch([0 0 1 1-e 0+e 0+e],[0 1 1 1-e 1-e 0+e],c3);plot([0 1 1 0 0],[0 0 1 1 0]);disp('W');
  "b{5}" : Constant  Value=0.08685313139123905512573031728607020340859889984130859375
      mask Display: e = 0.06;c1 = [120 150 230]/255;c2 = ([120 150 230]+0)/383;c3 = ([120 150 230]+128)/383;patch([0 1 1 0],[0 0 1 1],c1);patch([0 1 1 1-e 1-e 0+e],[0 0 1 1-e 0+e 0+e],c2);patch([0 0 1 1-e 0+e 0+e],[0 1 1 1-e 1-e 0+e],c3);plot([0 1 1 0 0],[0 0 1 1 0]);disp('b');
  netsum : Sum  Inputs=2  InputSameDT=on  SaturateOnIntegerOverflow=on  OutDataTypeStr=Inherit: Same as first input
      mask Display: e = 0.06;c1 = [120 150 230]/255;c2 = ([120 150 230]+0)/383;c3 = ([120 150 230]+128)/383;patch([0 1 1 0],[0 0 1 1],c1);patch([0 1 1 1-e 1-e 0+e],[0 0 1 1-e 0+e 0+e],c2);patch([0 0 1 1-e 0+e 0+e],[0 1 1 1-e 1-e 0+e],c3);plot([0 1 1 0 0],[0 0 1 1 0]);disp('+');
  purelin : neural/Transfer Functions/purelin
  "a{5}" : Outport  InitialOutput=0
      mask Display: e = 0.06;c1 = [120 230 180]/255;c2 = ([120 230 180]+0)/(256+128);c3 = ([120 230 180]+128)/(256+128);patch([0 1 1 0],[0 0 1 1],c1);patch([0 1 1 1-e 1-e 0+e],[0 0 1 1-e 0+e 0+e],c2);patch([0 0 1 1-e 0+e 0+e],[0 1 1 1-e 1-e 0+e],c3);plot([0 1 1 0 0],[0 0 1 1 0]);
  wires:
  purelin/1 -> "a{5}"/1
  netsum/1 -> purelin/1
  "b{5}"/1 -> netsum/2
  "LW{5,4}"/1("lz{5,4}") -> netsum/1
  Delays 1/1("pd{5,4}") -> "LW{5,4}"/1("ad{5,4}")
  "a{4} "/1 -> Delays 1/1("p{5}")

== system AFC_FFNN_trainbfg_15_15_15_15_Nor_July_15_RepFast/Air Fuel Control Model 1/Feed-Forward Neural Network/Process Input 1 ==
  x : Inport  PortDimensions=4
      mask Display: e = 0.06;c1 = [120 230 180]/255;c2 = ([120 230 180]+0)/(256+128);c3 = ([120 230 180]+128)/(256+128);patch([0 1 1 0],[0 0 1 1],c1);patch([0 1 1 1-e 1-e 0+e],[0 0 1 1-e 0+e 0+e],c2);patch([0 0 1 1-e 0+e 0+e],[0 1 1 1-e 1-e 0+e],c3);plot([0 1 1 0 0],[0 0 1 1 0]);
  p : Outport  PortDimensions=4
      mask Display: e = 0.06;c1 = [120 230 180]/255;c2 = ([120 230 180]+0)/(256+128);c3 = ([120 230 180]+128)/(256+128);patch([0 1 1 0],[0 0 1 1],c1);patch([0 1 1 1-e 1-e 0+e],[0 0 1 1-e 0+e 0+e],c2);patch([0 0 1 1-e 0+e 0+e],[0 1 1 1-e 1-e 0+e],c3);plot([0 1 1 0 0],[0 0 1 1 0]);
  wires:
  x/1 -> p/1

== system AFC_FFNN_trainbfg_15_15_15_15_Nor_July_15_RepFast/Air Fuel Control Model 1/Feed-Forward Neural Network/Process Output 1 ==
  a : Inport  PortDimensions=1
      mask Display: e = 0.06;c1 = [120 230 180]/255;c2 = ([120 230 180]+0)/(256+128);c3 = ([120 230 180]+128)/(256+128);patch([0 1 1 0],[0 0 1 1],c1);patch([0 1 1 1-e 1-e 0+e],[0 0 1 1-e 0+e 0+e],c2);patch([0 0 1 1-e 0+e 0+e],[0 1 1 1-e 1-e 0+e],c3);plot([0 1 1 0 0],[0 0 1 1 0]);
  y : Outport  PortDimensions=1
      mask Display: e = 0.06;c1 = [120 230 180]/255;c2 = ([120 230 180]+0)/(256+128);c3 = ([120 230 180]+128)/(256+128);patch([0 1 1 0],[0 0 1 1],c1);patch([0 1 1 1-e 1-e 0+e],[0 0 1 1-e 0+e 0+e],c2);patch([0 0 1 1-e 0+e 0+e],[0 1 1 1-e 1-e 0+e],c3);plot([0 1 1 0 0],[0 0 1 1 0]);
  wires:
  a/1 -> y/1

== system AFC_FFNN_trainbfg_15_15_15_15_Nor_July_15_RepFast/Air Fuel Control Model 1/Cylinder and Exhaust/A//F_sensor/Filter ==
  In : Inport
  Gain : Gain  Gain=50
  Integrator : Integrator  InitialCondition=14.7
  Sum : Sum  Inputs=|+-
  Out : Outport  VectorParamsAs1DForOutWhenUnconnected=off
  wires:
  Integrator/1 -> Out/1, Sum/2
  In/1 -> Sum/1
  Gain/1 -> Integrator/1
  Sum/1 -> Gain/1

== system AFC_FFNN_trainbfg_15_15_15_15_Nor_July_15_RepFast/Air Fuel Control Model 1/Feed-Forward Neural Network/Layer 1/Delays 1 ==
  "p{1}" : Inport  PortDimensions=4
      mask Display: e = 0.06;c1 = [120 230 180]/255;c2 = ([120 230 180]+0)/(256+128);c3 = ([120 230 180]+128)/(256+128);patch([0 1 1 0],[0 0 1 1],c1);patch([0 1 1 1-e 1-e 0+e],[0 0 1 1-e 0+e 0+e],c2);patch([0 0 1 1-e 0+e 0+e],[0 1 1 1-e 1-e 0+e],c3);plot([0 1 1 0 0],[0 0 1 1 0]);
  mux : Mux  Inputs=1
      mask Display: e = 0.06;c1 = [120 150 230]/255;c2 = ([120 150 230]+0)/383;c3 = ([120 150 230]+128)/383;patch([0 1 1 0],[0 0 1 1],c1);patch([0 1 1 1-e 1-e 0+e],[0 0 1 1-e 0+e 0+e],c2);patch([0 0 1 1-e 0+e 0+e],[0 1 1 1-e 1-e 0+e],c3);plot([0 1 1 0 0],[0 0 1 1 0]);disp('Mux')
  "pd{1,1}" : Outport
      mask Display: e = 0.06;c1 = [120 230 180]/255;c2 = ([120 230 180]+0)/(256+128);c3 = ([120 230 180]+128)/(256+128);patch([0 1 1 0],[0 0 1 1],c1);patch([0 1 1 1-e 1-e 0+e],[0 0 1 1-e 0+e 0+e],c2);patch([0 0 1 1-e 0+e 0+e],[0 1 1 1-e 1-e 0+e],c3);plot([0 1 1 0 0],[0 0 1 1 0]);
  wires:
  mux/1 -> "pd{1,1}"/1
  "p{1}"/1 -> mux/1
